simulink model "aircraft_Model"  (R2026b)
settings: Solver=ode1  StartTime=0  StopTime=100  FixedStep=0.01
values from neighbouring files (symbols this model uses):
  A_x = 10    [aircraft_parameter.m]
  c_dx = 0.3    [aircraft_parameter.m]
  c_L = 0.8    [aircraft_parameter.m]
  F_prop = 30000    [aircraft_parameter.m]
  g = 9.81    [aircraft_parameter.m]
  m = 5000    [aircraft_parameter.m]
  mu = 0.01    [aircraft_parameter.m]
  rho_A = 1.2    [aircraft_parameter.m]
settings Model: Creator=at  LastModifiedBy=at

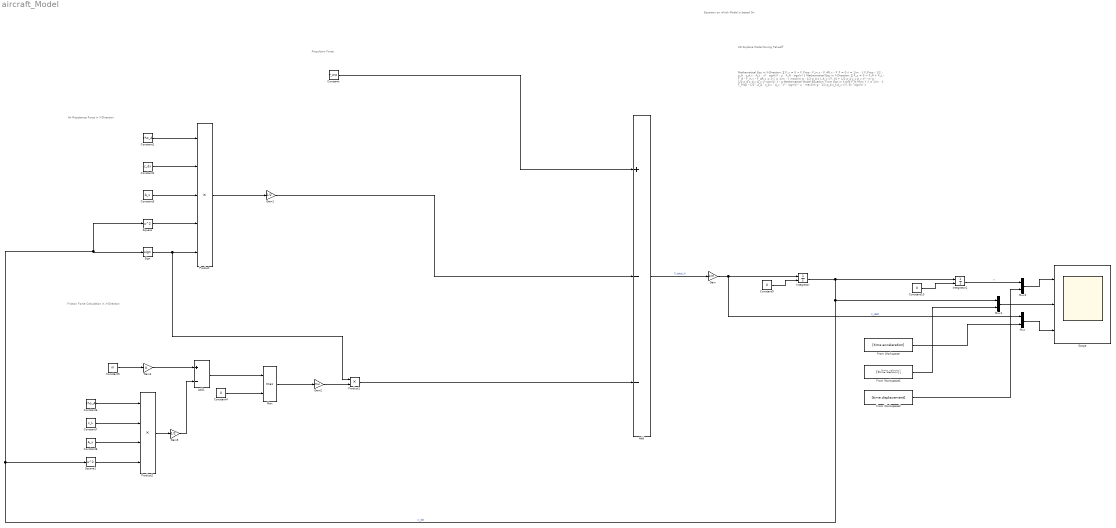
== system aircraft_Model ==
  note: Equation on which Model is based On
  note: Mathematical Equ in X-Direction:
      | ∑ F_x = 0 ⇒ F_Prop - F_in,x - F_AR,x - F_F = 0
      |
      | ẍ = 1/m · { F_Prop - 1/2 · ρ_A · c_d,x · A_x · ẋ² · sign(ẋ) - μ · F_N · sign(ẋ) }
      |
      | Mathematical Equ in Y-Direction:
      | ∑ F_y = 0 ⇒ F_N + F_L - F_G - F_in,y - F_AR,y = 0
      |
      | ÿ = 1/m · { max[(m·g - 1/2·ρ_A·c_L·A_x·ẋ²), 0] + 1/2·ρ_A·c_L·A_x·ẋ² - m·g - 1/2·ρ_A·c_d,y·A_y·ẏ²·sign(ẏ) } - g
      |
      | Mathematical Model Equation: From Eqn in X and F_N from Y
      |
      | ẍ = 1/m · { F_Prop - 1/2 · ρ_A · c_d,x · A_x · ẋ² · sign(ẋ) - μ · max[(m·g - 1/2·ρ_A·c_L·A_x·ẋ²), 0] · sign(ẋ) }
  note: 2D Airplane Model During Takeoff
  note: [time velocity]
  note: Propulsion Force
  note: Friction Force Calculation in X-Direction
  note: Air Resistance Force in X-Direction
  Add : Sum  Inputs=+--
  Add1 : Sum  Inputs=+-
  Constant : Constant  Value=F_prop
      settings: AttributesFormatString=Propulsion: %<Value>
  Constant1 : Constant  Value=rho_A
      settings: AttributesFormatString=%<Value> [kg/m^3]
  Constant10 : Constant  Value=0
      settings: AttributesFormatString=%<Value> [m/s]
  Constant2 : Constant  Value=c_dx
      settings: AttributesFormatString=%<Value> [-]
  Constant3 : Constant  Value=A_x
      settings: AttributesFormatString=%<Value> [m^2]
  Constant4 : Constant  Value=0
  Constant5 : Constant  Value=m
      settings: AttributesFormatString=%<Value> [kg]
  Constant6 : Constant  Value=rho_A
      settings: AttributesFormatString=%<Value> [kg/m^3]
  Constant7 : Constant  Value=c_L
      settings: AttributesFormatString=%<Value> [-]
  Constant8 : Constant  Value=A_x
      settings: AttributesFormatString=%<Value> [m^2]
  Constant9 : Constant  Value=0
      settings: AttributesFormatString=%<Value> [m/s^2]
  From Workspace : FromWorkspace  VariableName=[time acceleration]
  From Workspace1 : FromWorkspace  VariableName=[time velocity]
  From Workspace2 : FromWorkspace  VariableName=[time displacement]
  Gain : Gain  Gain=1/m
      settings: AttributesFormatString=Gain:%<Gain>
  Gain1 : Gain  Gain=1/2
      settings: AttributesFormatString=Gain%<Gain>
  Gain2 : Gain  Gain=mu
      settings: AttributesFormatString=%<Gain> [-]
  Gain4 : Gain  Gain=g
      settings: AttributesFormatString=%<Gain> [m/s^2]
  Gain5 : Gain  Gain=1/2
      settings: AttributesFormatString=%<Gain> [-]
  Integrator : Integrator  InitialConditionSource=external
  Integrator1 : Integrator  InitialConditionSource=external
  Max : MinMax  Function=max  Inputs=2
  Mux : Mux  Inputs=2
  Mux1 : Mux  Inputs=2
  Mux2 : Mux  Inputs=2
  Product : Product  Inputs=5
  Product1 : Product
  Product2 : Product  Inputs=4
  Scope : Scope  NumInputPorts=3
      settings: ActiveDisplayYMinimum=-1370.3493057816618  ActiveDisplayYMaximum=12333.143752034957
  Sign : Signum
  Square : Math  Operator=square
  Square1 : Math  Operator=square
  wires:
  Gain/1 -> Mux/1, Integrator/1  "X_ddot"
  Integrator/1 -> Mux1/1, Sign/1, Square/1, Square1/1, Integrator1/1  "X_dot"
  Integrator1/1 -> Mux2/1  "x"
  Add/1 -> Gain/1  "F_total_N"
  Constant/1 -> Add/1
  Gain1/1 -> Add/2
  Product/1 -> Gain1/1
  Constant1/1 -> Product/1
  Constant2/1 -> Product/2
  Constant3/1 -> Product/3
  Square/1 -> Product/4
  Sign/1 -> Product1/1, Product/5
  Max/1 -> Gain2/1
  Gain2/1 -> Product1/2
  Product1/1 -> Add/3
  Add1/1 -> Max/1
  Constant4/1 -> Max/2
  Gain4/1 -> Add1/1
  Constant5/1 -> Gain4/1
  Constant8/1 -> Product2/3
  Constant7/1 -> Product2/2
  Product2/1 -> Gain5/1
  Gain5/1 -> Add1/2
  Constant6/1 -> Product2/1
  Square1/1 -> Product2/4
  Constant9/1 -> Integrator/2
  Constant10/1 -> Integrator1/2
  From Workspace/1 -> Mux/2
  From Workspace2/1 -> Mux2/2
  From Workspace1/1 -> Mux1/2
  Mux1/1 -> Scope/2
  Mux/1 -> Scope/3
  Mux2/1 -> Scope/1
